simulink model "D1_f"  (R2026b)
settings: Solver=ode4  StopTime=20  FixedStep=1e-3
settings Model: Creator=User  LastModifiedBy=20251710

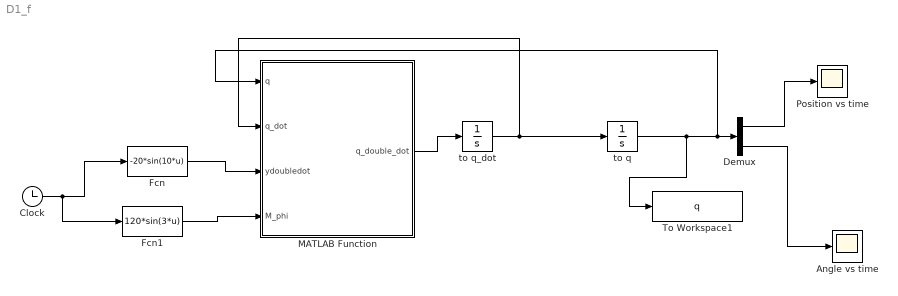
== system D1_f ==
  Angle vs time : Scope
      settings: Title=Milling head angle  ActiveDisplayYMinimum=-4.3009128120502655  ActiveDisplayYMaximum=2.1218248156626718  YLabel=\phi [rad]
  Clock : Clock
      settings: Decimation=20
  Demux : Demux  Outputs=2
  Fcn : Fcn  Expr=-20*sin(10*u)
  Fcn1 : Fcn  Expr=120*sin(3*u)
  MATLAB Function : MATLAB Function  TreatAsAtomicUnit=on
  Position vs time : Scope
      settings: Title=Carriage position  ActiveDisplayYMinimum=-0.052715362460519666  ActiveDisplayYMaximum=0.91128643071953919  YLabel=x [m]
  To Workspace1 : ToWorkspace  VariableName=q  SampleTime=-1
  to q : Integrator  InitialCondition=[0.1, -pi/4]
  to q_dot : Integrator  InitialCondition=[0,0]
  wires:
  Demux/1 -> Position vs time/1
  to q_dot/1 -> MATLAB Function/2(q_dot), to q/1
  to q/1 -> To Workspace1/1, MATLAB Function/1(q), Demux/1
  MATLAB Function/1(q_double_dot) -> to q_dot/1
  Demux/2 -> Angle vs time/1
  Fcn/1 -> MATLAB Function/3(ydoubledot)
  Fcn1/1 -> MATLAB Function/4(M_phi)
  Clock/1 -> Fcn1/1, Fcn/1

== matlab function D1_f/MATLAB Function ==
  data: q input; q_double_dot output; q_dot input; ydoubledot input; M_phi input
function q_double_dot = fcn(q,q_dot, ydoubledot, M_phi)


%constants
g=-9.81;
L23=0.05;
mh=0.7;
mc=2;
phi_h3=2*pi/3;
xPDref=0.5;
kPD=380;
k_phi=100;
phi_ref=-pi/2;
dPD=10;
dx=0.5;
d_phi=2;
Jh2=1.2;




%Generalised coordinates
x=q(1);
phi=q(2);

xdot=q_dot(1);
phi_dot=q_dot(2);

%solution


M=[ (mh+mc) , -mh*L23*sin(phi-phi_h3);
    -mh*L23*sin(phi-phi_h3) , Jh2
    ];

F=[-(dPD+dx)*xdot + (mh*L23*cos(phi-phi_h3))*(phi_dot^2) - kPD*(x-xPDref);
   M_phi-(d_phi*phi_dot) - mh*L23*(ydoubledot+g)*cos(phi-phi_h3) - k_phi*(phi-phi_ref) 
];

q_double_dot=transpose(M\F);
